simulink model "quantization"  (Simulink 4.00)
settings: Solver=ode45  StartTime=0.0  StopTime=10.0  RelTol=1e-3
libraries: simulink_extras x1
settings Model: Creator=mcar  LastModifiedBy=mcar  BlockReductionOpt=off

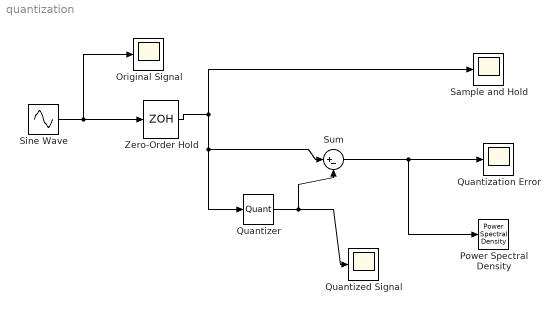
== system quantization ==
  Original Signal : Scope
      settings: TimeRange=auto  YMin=-5  YMax=5  SaveToWorkspace=off  SaveName=ScopeData3  LimitDataPoints=on  MaxDataPoints=5000
  Power Spectral Density : simulink_extras/Additional Sinks/Power Spectral Density  npts=128  fftpts=512  HowOften=64  sampleT=0.1
  Quantization Error : Scope
      settings: TimeRange=auto  YMin=-5  YMax=5  SaveToWorkspace=off  SaveName=ScopeData2  LimitDataPoints=on  MaxDataPoints=5000
  Quantized Signal : Scope
      settings: TimeRange=auto  YMin=-5  YMax=5  SaveToWorkspace=off  LimitDataPoints=on  MaxDataPoints=5000
  Quantizer : Quantizer  QuantizationInterval=.1  LinearizeAsGain=on
  Sample and Hold : Scope
      settings: TimeRange=auto  YMin=-5  YMax=5  SaveToWorkspace=off  SaveName=ScopeData  LimitDataPoints=on  MaxDataPoints=5000
  Sine Wave : Sin  Amplitude=10  Frequency=1  Phase=0  SampleTime=0
  Sum : Sum  Inputs=|+-  SaturateOnIntegerOverflow=on
  Zero-Order Hold : ZeroOrderHold  SampleTime=.1
  wires:
  Sine Wave/1 -> Zero-Order Hold/1, Original Signal/1
  Zero-Order Hold/1 -> Sample and Hold/1, Quantizer/1, Sum/1
  Quantizer/1 -> Quantized Signal/1, Sum/2
  Sum/1 -> Quantization Error/1, Power Spectral Density/1
